simulink model "xz_packaging_automatic"  (R2025b)
settings: Solver=ode15s  StartTime=0.0  StopTime=10.45  MaxStep=0.001  RelTol=1e-6  AbsTol=1e-9
model workspace: external: MATLAB File xz_packaging_automatic_DataFile.m (data not in the file)
values from neighbouring files (symbols this model uses):
  payloadMass_kg = 0.25    [xz_packaging_automatic_DataFile.m]
undefined symbols (not defined in the file or in its folder): smiData, X, Y, Z
libraries: sm_lib x2549, nesl_utility x31
(part 38 of 38)

== matlab function xz_packaging_automatic/Vacuum interlocks ==
  data: t input; stage output; dL input; dR input; fL input; fR input; process input; start output; pressure output; owner output; vacuum output; seat output; q input; v input; travel input; cycle output; holdPose output; stations output; axisReference input
function [stage,start,pressure,owner,vacuum,seat,cycle,holdPose,stations] = automatic_process(t,dL,dR,fL,fR,process,q,v,travel,axisReference)
% process = [start stop reset supplyCarton supplyCarrier unload leak inReady outReady axesReady ventBlocked settlePermit].
% Travel uses positive process direction on each belt.
% 1 ms bench interlock. Owner: 1 = infeed, 2 = tool, 3 = outfeed.
persistent phase entered dp readySince count fault last seen fed carried hold holdVac base parked followingSince
if isempty(phase)
    phase = 0;
    entered = 0;
    dp = zeros(2,1);
    readySince = -1;
    count = 0;
    fault = 0;
    last = zeros(5,1);
    seen = false(2,1);
    fed = false;
    carried = 1;
    hold = [0.05;0.024;0;0];
    holdVac = false;
    base = zeros(2,1);
    parked = false;
    followingSince = -1;
end
elapsed = t-entered;
process = process(:);
rising = process([1 3 4 5 6])>0.5 & last<=0.5;
last = process([1 3 4 5 6]);
registered = fed && abs(travel(2)-base(2)-0.015)<=0.0005;
productAtPick = fed && abs(travel(1)-base(1)-0.16)<=0.0005;
leakRight = process(7);
atPick = abs(q(1)-0.05)<=0.00005;
atDrop = abs(q(1)-0.45)<=0.00005;
seatLeft = dL>=0.0005 && dL<=0.002 && fL>2;
seatRight = dR>=0.0005 && dR<=0.002 && fR>2;
seat = seatLeft && seatRight && fL+fR<=10;
energized = phase>=2 && phase<=7 || (phase==90 && holdVac);
holdingSeal = phase>=3 && phase<=7 || (phase==90 && holdVac);
target = zeros(2,1);
tau = 0.06;
if energized
    target = 5000 + 55000*double([seatLeft || holdingSeal; seatRight || holdingSeal]);
    if leakRight > 0.5
        target(2) = min(target(2),25000);
    end
    tau = 0.10;
end
if t > 0 && ~(phase==8 && process(11)>0.5) && ~(phase==90 && fault==4)
    dp = target + (dp-target)*exp(-0.001/tau);
end
motion = [0.28499999999999998 2.6499999999999999 0.055 0.67658225753061907;0.28499999999999998 2.6499999999999999 0.055 0.68886295928500485;0.57999999999999996 2.3999999999999999 0.055 0.98632183908045978;0.0067999999999999996 0.16 0.02 0.79779411764705888;0.0085000000000000006 0.16 0.02 0.48488970588235292;0.0067999999999999996 0.16 0.02 0.2830882352941177];
next = phase;
stopped = all(abs(v)<=0.005);
raised = abs(q(2)-0.024)<=0.00005;
atHome = atPick && raised && stopped;
ready = false;
switch phase
    case 1
        ready = elapsed>=motion(1,4)+motion(4,4) && atPick && abs(q(2)-0.1755)<=0.00005 && stopped;
    case 3
        ready = elapsed>=0.30 && atPick && abs(q(2)-0.174)<=0.00005 && stopped;
    case 4
        ready = elapsed>=motion(2,4) && atPick && abs(q(2)-0.024)<=0.00005 && stopped;
    case 5
        ready = elapsed>=motion(3,4) && atDrop && registered && abs(q(2)-0.024)<=0.00005 && stopped;
    case 6
        ready = elapsed>=motion(1,4)+motion(5,4) && atDrop && registered && abs(q(2)-0.174)<=0.00005 && stopped;
    case 7
        ready = elapsed>=motion(6,4) && atDrop && registered && seat && abs(q(2)-0.1755)<=0.00005 && stopped;
    case 9
        ready = elapsed>=0.30+motion(2,4) && atDrop && abs(q(2)-0.024)<=0.00005 && stopped;
    case 21
        ready = elapsed>=1 && abs(travel(1)-base(1)-0.16)<=0.0005 && ...
            abs(travel(2)-base(2)-0.015)<=0.0005 && atHome;
    case 22
        ready = elapsed>=1 && abs(travel(2)-base(2)-0.175)<=0.0005 && atDrop && raised && stopped;
    case 23
        ready = elapsed>=motion(3,4) && atHome;
    case 12
        ready = elapsed>=1.30 && atPick && abs(q(2)-0.024)<=0.00005 && stopped;
end
ready = ready && (phase==21 || phase==22 || process(12)>0.5);
if ~ready
    readySince = -1;
elseif readySince<0
    readySince = t;
end
settled = readySince>=0 && t-readySince>=0.05;
switch phase
    case 0
        if rising(1) && atHome && process(10)>0.5
            next = 20;
        end
    case 20
        seen = seen | rising(3:4);
        if all(seen) && atHome && process(10)>0.5
            next = 21;
            fed = true;
            parked = false;
        end
    case 21
        if settled
            next = 1;
        elseif elapsed>=1.60
            fault = 2;
        end
    case 1
        if settled
            next = 2;
        end
    case 2
        if seat && atPick && productAtPick && elapsed>=0.10 && all(dp>=58000)
            next = 3;
        elseif elapsed>=0.60
            next = 11;
            fault = 1;
        end
    case 3
        if settled
            next = 4;
        end
    case 4
        if settled
            next = 5;
        end
    case 5
        if settled
            next = 6;
        end
    case 6
        if settled
            next = 7;
        end
    case 7
        if settled
            next = 8;
        elseif elapsed>=1.20
            fault = 3;
        end
    case 8
        if ~registered || ~atDrop || ~seat
            fault = 3;
        elseif elapsed>=0.08 && all(dp<=5000) && process(2)<=0.5 && process(10)>0.5
            next = 9;
            count = count+1;
        elseif elapsed>=0.50
            fault = 4;
        end
    case 9
        if settled
            next = 22;
        end
    case 22
        if settled
            next = 24;
        elseif elapsed>=1.60
            fault = 2;
        end
    case 24
        if rising(5)
            next = 23;
        elseif elapsed>=2.0
            fault = 5;
        end
    case 23
        if settled
            next = 20;
            base = base+[0.16;0.175];
            fed = false;
            seen(:) = false;
            parked = true;
        end
    case 13
        if rising(2) && atHome && ~any(process(4:5)>0.5)
            next = 0;
            fault = 0;
            fed = false;
            base = travel;
            seen(:) = false;
        end
    case 90
        if rising(2) && atHome && carried==1 && ~holdVac && ~any(process(4:5)>0.5)
            next = 0;
            fault = 0;
            fed = false;
            base = travel;
            seen(:) = false;
        end
    case 11
        if all(dp<=5000)
            next = 12;
        end
    case 12
        if settled
            next = 13;
        end
end
axisTimeout = (phase==1 && elapsed>2.65) || (phase==3 && elapsed>0.80) || ...
    (phase==4 && elapsed>1.50) || (phase==5 && elapsed>1.80) || ...
    (phase==6 && elapsed>2.30) || (phase==7 && elapsed>1.20) || ...
    ((phase==9 || phase==12 || phase==23) && elapsed>1.80);
axisMoving = any(phase==[1 3 4 5 6 7 9 12 23]);
if axisMoving && any(abs(q-axisReference(:,1))>0.002)
    if followingSince<0
        followingSince = t;
    end
else
    followingSince = -1;
end
if phase~=90 && phase~=13
    if process(2)>0.5
        fault = 6;
    elseif process(10)<=0.5 && phase~=0 && phase~=20 || axisTimeout
        fault = 3;
    elseif (phase==21 || phase==22) && abs(q(2)-0.024)>0.0005
        fault = 3;
    elseif phase>=4 && phase<=6 && any(dp<58000)
        fault = 7;
    elseif followingSince>=0 && t-followingSince>=0.020
        fault = 8;
    end
    if fault~=0 && (fault~=1 || axisTimeout)
        next = 90;
        hold = [q;travel];
        carried = ownership(phase,parked);
        holdVac = phase>=2 && phase<=7;
    end
end
if next~=phase
    phase = next;
    entered = t;
    readySince = -1;
end
stage = phase;
start = entered;
pressure = dp;
owner = ownership(stage,parked);
if stage==90
    owner = carried;
end
vacuum = double(stage>=2 && stage<=7 || (stage==90 && holdVac));
cycle = [count;fault;double(stage==20 && count>0);base;double(fed); ...
    double(process(8)>0.5);double(process(9)>0.5);double(parked)];
holdPose = hold;
stations = [double(productAtPick);double(registered);travel(2)-base(2)-0.015;leakRight];
end

function owner = ownership(stage,parked)
owner = 1;
if stage>=4 && stage<=6
    owner = 2;
elseif (stage>=7 && stage<=9) || any(stage==[22 23 24]) || (stage==20 && parked)
    owner = 3;
end
end

== matlab function xz_packaging_automatic/Bench trajectory reference ==
  data: t input; x output; stage input; start input; z output; cycle input; holdPose input; owner input; belts output; cartonY output; carrierY output
function [x,z,belts,cartonY,carrierY] = automatic_reference(t,stage,start,cycle,holdPose,owner)
% Rows are position (m), velocity (m/s), acceleration (m/s^2).
% X travel is positive world X. Tool Z travel is positive down.
motion = [0.28499999999999998 2.6499999999999999 0.055 0.67658225753061907;0.28499999999999998 2.6499999999999999 0.055 0.68886295928500485;0.57999999999999996 2.3999999999999999 0.055 0.98632183908045978;0.0067999999999999996 0.16 0.02 0.79779411764705888;0.0085000000000000006 0.16 0.02 0.48488970588235292;0.0067999999999999996 0.16 0.02 0.2830882352941177];
dt = t-start;
x = [0.05;0;0];
z = [0.1755;0;0];
switch stage
    case {0,20,21}
        z(1) = 0.024;
    case 1
        if dt < motion(1,4)
            z = phase8_stroke(dt,motion(1,:),0.024,0.1705);
        else
            z = phase8_stroke(dt-motion(1,4),motion(4,:),0.1705,0.1755);
        end
    case 3
        z = stroke(dt,0.30,0.1755,0.174);
    case 4
        z = phase8_stroke(dt,motion(2,:),0.174,0.024);
    case 5
        z(1) = 0.024;
        x = phase8_stroke(dt,motion(3,:),0.05,0.45);
    case 6
        x(1) = 0.45;
        if dt < motion(1,4)
            z = phase8_stroke(dt,motion(1,:),0.024,0.1705);
        else
            z = phase8_stroke(dt-motion(1,4),motion(5,:),0.1705,0.174);
        end
    case 7
        x(1) = 0.45;
        z = phase8_stroke(dt,motion(6,:),0.174,0.1755);
    case {8,14}
        x(1) = 0.45;
    case {9,12}
        if stage == 9
            x(1) = 0.45;
        end
        if dt < 0.30
            z = stroke(dt,0.30,0.1755,0.174);
        elseif stage == 9
            z = phase8_stroke(dt-0.30,motion(2,:),0.174,0.024);
        else
            z = stroke(dt-0.30,1,0.174,0.024);
        end
    case {22,24}
        x(1) = 0.45;
        z(1) = 0.024;
    case 23
        x = phase8_stroke(dt,motion(3,:),0.45,0.05);
        z(1) = 0.024;
    case 13
        z(1) = 0.024;
    case 90
        x(1) = holdPose(1);
        z(1) = holdPose(2);
end
base = cycle(4:5);
in = [base(1);0;0];
out = [base(2);0;0];
if stage==21
    in = stroke(dt,1,base(1),base(1)+0.16*cycle(7));
    out = stroke(dt,1,base(2),base(2)+0.015*cycle(8));
elseif any(stage==[1:9 11:13 22:24])
    in(1) = base(1)+0.16;
    out(1) = base(2)+0.015;
    if stage==22
        out = stroke(dt,1,out(1),out(1)+0.16*cycle(8));
    elseif stage==23 || stage==24
        out(1) = out(1)+0.16;
    end
elseif stage==90
    in(1) = holdPose(3);
    out(1) = holdPose(4);
end
belts = [in;out];
carrierY = out-[base(2)+0.015;0;0];
if stage==20 && cycle(9)>0.5
    carrierY = [0.16;0;0];
end
cartonY = [base(1)+0.16;0;0]-in;
if owner==2
    cartonY = zeros(3,1);
elseif owner==3
    cartonY = carrierY;
end

end

function y = stroke(t,duration,first,last)
s = min(1,max(0,t/duration));
d = last-first;
y = [first+d*s^3*(10-15*s+6*s^2); ...
     d/duration*30*s^2*(1-s)^2; ...
     d/duration^2*60*s*(1-s)*(1-2*s)];
end


function y = phase8_stroke(t,profile,first,last)
%#codegen
speed = profile(1);
acceleration = profile(2);
ramp = profile(3);
total = profile(4);
if t<=0
    y = [first;0;0];
    return
elseif t>=total
    y = [last;0;0];
    return
end
holdAcceleration = speed/acceleration-ramp;
cruise = total-2*(holdAcceleration+2*ramp);
duration = [ramp holdAcceleration ramp cruise ramp holdAcceleration ramp];
jerk = (acceleration/ramp)*[1 0 -1 0 -1 0 1];
position = 0;
velocity = 0;
accel = 0;
for k = 1:7
    dt = min(t,duration(k));
    j = jerk(k);
    position = position+velocity*dt+0.5*accel*dt^2+j*dt^3/6;
    velocity = velocity+accel*dt+0.5*j*dt^2;
    accel = accel+j*dt;
    t = t-dt;
end
y = [first;0;0]+sign(last-first)*[position;velocity;accel];
end

== matlab function xz_packaging_automatic/Carton coupling ==
  data: owner input; cx output; q input; v input; a input; process input; cz output; load output; required output; contact output; payload input
function [cx,cz,load,required,contact] = carton_coupling(owner,q,v,a,process,payload)
% The carton is constrained to the tool only while carried.
cx = zeros(3,1);
cz = zeros(3,1);
load = zeros(3,1);
required = 0;
contact = double((owner==1 && process(1)>0.5 && abs(q(1)-0.05)<0.0005) || ...
    (owner==3 && process(2)>0.5 && abs(process(3))<=0.0005 && abs(q(1)-0.45)<0.0005));
if owner==2
    cx = [q(1)-0.05;v(1);a(1)];
    cz = [max(0,0.174-q(2));-v(2);-a(2)];
    load = payload*[a(1);0;9.80665-a(2)];
    moment = abs(load(1))*0.015+load(3)*0.002;
    required = 2*(load(3)/2+moment/0.036+abs(load(1))/(2*0.30));
elseif owner==3
    cx(1) = 0.4;
end
end
